simulink model "snap_adc5g_spec_rpi"  (R2019a)
settings: Solver=VariableStepDiscrete  StartTime=0.0  StopTime=10.0  RelTol=1e-3
undefined symbols (not defined in the file): pfb_coeff_gen_calc
libraries: xbsIndex_r4 x13965, casper_library_misc x80, casper_library_delays x43, xps_library x5, xbsReplacements_r4 x2, casper_library_communications x1
(part 3 of 152)

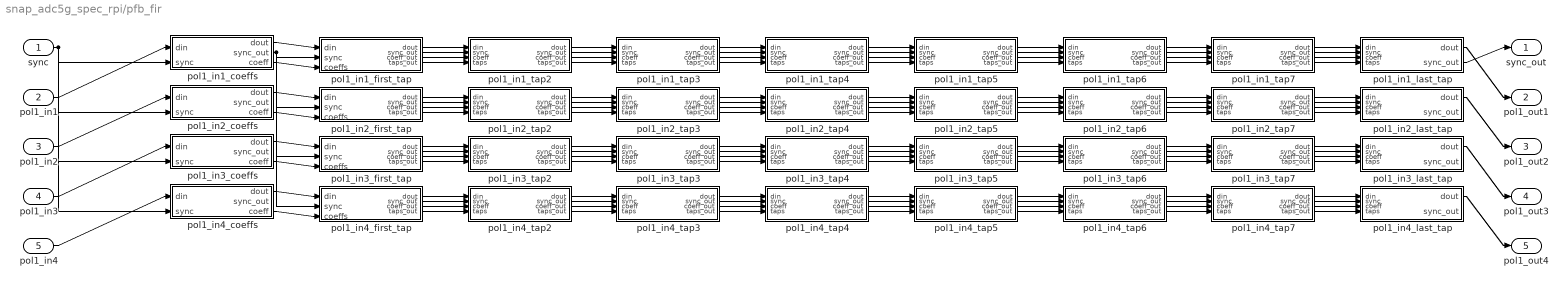
== system snap_adc5g_spec_rpi/pfb_fir ==
  sync : Inport
  pol1_in1 : Inport  Port=2
  pol1_in2 : Inport  Port=3
  pol1_in3 : Inport  Port=4
  pol1_in4 : Inport  Port=5
  pol1_in1_coeffs : Subsystem  AncestorBlock=casper_library_pfbs/pfb_coeff_gen  mask(pfb_coeff_gen){PFBSize=13, CoeffBitWidth=18, TotalTaps=8, CoeffDistMem=off, WindowType=hamming, bram_latency=3, n_inputs=2, nput=0, fwidth=1, debug_mode=off, fan_latency=1}
      mask prompts: PFBSize "Size of PFB: (2^? pnts)"; CoeffBitWidth "Bitwidth of Coefficients:"; TotalTaps "Total Number of Taps:"; CoeffDistMem "Implement Coeff Gen in Distributed Memory"; WindowType "Windowing Function:"; bram_latency "BRAM Latency"; n_inputs "Number of Simultaneous Inputs: (2^?)"; nput "This is input number:"; fwidth "Bin Width (normal=1)"; debug_mode "Debug mode - coeffs are a [1:pfb_size*taps] ramp."; fan_latency "Fanout latency"
      mask init:
      | pfb_coeff_gen_init(gcb, ...
      |     'PFBSize', PFBSize, ...
      |     'CoeffBitWidth', CoeffBitWidth, ...
      |     'TotalTaps', TotalTaps, ...
      |     'CoeffDistMem', CoeffDistMem, ...
      |     'WindowType', WindowType, ...
      |     'bram_latency', bram_latency, ...
      |     'n_inputs', n_inputs, ...
      |     'nput', nput, ...
      |     'fwidth', fwidth, ...
      |     'fan_latency', fan_latency, ...
      |     'debug_mode', debug_mode);
      settings: AttributesFormatString=|
      | PFBSize=13, n_inputs=2,
      | taps=8, input=0
  pol1_in1_first_tap : Subsystem  AncestorBlock=casper_library_pfbs/first_tap  mask(first_tap){PFBSize=13, CoeffBitWidth=18, TotalTaps=8, BitWidthIn=8, WindowType=hamming, mult_latency=2, bram_latency=3, n_inputs=2, fwidth=1, use_hdl=on, use_embedded=off}
      mask prompts: PFBSize "Size of PFB: (2^? pnts)"; CoeffBitWidth "Bitwidth of Coefficients:"; TotalTaps "Total Number of Taps:"; BitWidthIn "Input Bitwidth:"; WindowType "Windowing Function:"; mult_latency "Mult Latency"; bram_latency "BRAM Latency"; n_inputs "Number of Simultaneous Inputs: (2^?)"; fwidth "Bit Width (normal=1)"; use_hdl "Use behavioral HDL for multlipliers"; use_embedded "Use embedded multipliers"
      mask init:
      | first_tap_init(gcb,...
      |     'PFBSize', PFBSize,...
      |     'CoeffBitWidth', CoeffBitWidth,...
      |     'TotalTaps', TotalTaps,...
      |     'BitWidthIn', BitWidthIn,...
      |     'WindowType', WindowType,...
      |     'mult_latency', mult_latency,...
      |     'bram_latency', bram_latency,...
      |     'n_inputs', n_inputs,...
      |     'fwidth', fwidth,...
      |     'use_hdl', use_hdl,...
      |     'use_embedded', use_embedded);
      settings: AttributesFormatString=taps=8
      mask TypeOptions WindowType: bartlett | barthannwin | blackman | blackmanharris | bohamwin | chebwin | flattopwin | gausswin | hamming | hann | kaiser | nuttallwin | parzenwin | rectwin | tukeywin | triang
      mask Callback use_hdl:
      | use_hdl = get_param(gcb,'use_hdl');
      | if( strcmp(use_hdl,'on')),
      |     set_param(gcb, 'use_embedded','off');
      |     set_param(gcb, 'MaskVisibilities',{'on','on','on','on','on','on','on','on','on','on','off'});
      | else,
      |     set_param(gcb, 'MaskVisibilities',{'on','on','on','on','on','on','on','on','on','on','on'});
      | end
  pol1_in1_last_tap : Subsystem  AncestorBlock=casper_library_pfbs/last_tap  mask(last_tap){TotalTaps=8, BitWidthIn=8, BitWidthOut=18, CoeffBitWidth=18, add_latency=1, mult_latency=2, quantization=Round  (unbiased: Even Values), use_hdl=on, use_embedded=off}
      mask prompts: TotalTaps "Total Number of Taps:"; BitWidthIn "Input Bitwidth:"; BitWidthOut "Output Bitwidth:"; CoeffBitWidth "Coeff Bitwidth:"; add_latency "Add Latency"; mult_latency "Mult Latency"; quantization "Quantization Behavior"; use_hdl "Use behavioral HDL for multlipliers"; use_embedded "Use embedded multipliers"
      mask init:
      | last_tap_init(gcb,...
      |     'TotalTaps', TotalTaps,...
      |     'BitWidthIn', BitWidthIn,...
      |     'BitWidthOut', BitWidthOut,...
      |     'CoeffBitWidth', CoeffBitWidth,...
      |     'add_latency', add_latency,...
      |     'mult_latency', mult_latency,...
      |     'quantization', quantization,...
      |     'use_hdl', use_hdl,...
      |     'use_embedded', use_embedded);
      settings: AttributesFormatString=taps=8
      mask TypeOptions quantization: Truncate | Round  (unbiased: +/- Inf) | Round  (unbiased: Even Values)
      mask Callback use_hdl:
      | use_hdl = get_param(gcb,'use_hdl');
      | if( strcmp(use_hdl,'on')),
      |     set_param(gcb, 'use_embedded','off');
      |     set_param(gcb, 'MaskVisibilities',{'on','on','on','on','on','on','on','on','off'});
      | else,
      |     set_param(gcb, 'MaskVisibilities',{'on','on','on','on','on','on','on','on','on'});
      | end
  pol1_in1_tap2 : Subsystem  AncestorBlock=casper_library_pfbs/tap  mask(tap){mult_latency=2, coeff_width=18, coeff_frac_width=17, delay=2048, data_width=8, bram_latency=3, use_hdl=on, use_embedded=off}
      mask prompts: mult_latency "Multiplier Latency"; coeff_width "Coefficient Bit Width In"; coeff_frac_width "Coefficient Fractional Bits"; delay "Data/Sync Delay"; data_width "Data Bit Width In"; bram_latency "BRAM Latency"; use_hdl "Use behavioral HDL for multlipliers"; use_embedded "Use embedded multipliers"
      mask init:
      | use_hdl = get_param(gcb,'use_hdl');
      | use_embedded = get_param(gcb,'use_embedded');
      | set_param(gcb,'LinkStatus','inactive');
      | 
      | set_param([gcb,'/Mult'],'use_embedded',use_embedded);
      | set_param([gcb,'/Mult'],'use_behavioral_HDL',use_hdl);
      | set_param([gcb,'/Mult1'],'use_embedded',use_embedded);
      | set_param([gcb,'/Mult1'],'use_behavioral_HDL',use_hdl);
      mask Callback use_hdl:
      | use_hdl = get_param(gcb,'use_hdl');
      | if( strcmp(use_hdl,'on')),
      |     set_param(gcb, 'use_embedded','off');
      |     set_param(gcb, 'MaskVisibilities',{'on','on','on','on','on','on','on','off'});
      | else,
      |     set_param(gcb, 'MaskVisibilities',{'on','on','on','on','on','on','on','on'});
      | end
  pol1_in1_tap3 : Subsystem  AncestorBlock=casper_library_pfbs/tap  mask(tap){mult_latency=2, coeff_width=18, coeff_frac_width=17, delay=2048, data_width=8, bram_latency=3, use_hdl=on, use_embedded=off}
      mask prompts: mult_latency "Multiplier Latency"; coeff_width "Coefficient Bit Width In"; coeff_frac_width "Coefficient Fractional Bits"; delay "Data/Sync Delay"; data_width "Data Bit Width In"; bram_latency "BRAM Latency"; use_hdl "Use behavioral HDL for multlipliers"; use_embedded "Use embedded multipliers"
      mask init: same as snap_adc5g_spec_rpi/pfb_fir/pol1_in1_tap2
      mask Callback use_hdl:
      | use_hdl = get_param(gcb,'use_hdl');
      | if( strcmp(use_hdl,'on')),
      |     set_param(gcb, 'use_embedded','off');
      |     set_param(gcb, 'MaskVisibilities',{'on','on','on','on','on','on','on','off'});
      | else,
      |     set_param(gcb, 'MaskVisibilities',{'on','on','on','on','on','on','on','on'});
      | end
  pol1_in1_tap4 : Subsystem  AncestorBlock=casper_library_pfbs/tap  mask(tap){mult_latency=2, coeff_width=18, coeff_frac_width=17, delay=2048, data_width=8, bram_latency=3, use_hdl=on, use_embedded=off}
      mask prompts: mult_latency "Multiplier Latency"; coeff_width "Coefficient Bit Width In"; coeff_frac_width "Coefficient Fractional Bits"; delay "Data/Sync Delay"; data_width "Data Bit Width In"; bram_latency "BRAM Latency"; use_hdl "Use behavioral HDL for multlipliers"; use_embedded "Use embedded multipliers"
      mask init: same as snap_adc5g_spec_rpi/pfb_fir/pol1_in1_tap2
      mask Callback use_hdl:
      | use_hdl = get_param(gcb,'use_hdl');
      | if( strcmp(use_hdl,'on')),
      |     set_param(gcb, 'use_embedded','off');
      |     set_param(gcb, 'MaskVisibilities',{'on','on','on','on','on','on','on','off'});
      | else,
      |     set_param(gcb, 'MaskVisibilities',{'on','on','on','on','on','on','on','on'});
      | end
  pol1_in1_tap5 : Subsystem  AncestorBlock=casper_library_pfbs/tap  mask(tap){mult_latency=2, coeff_width=18, coeff_frac_width=17, delay=2048, data_width=8, bram_latency=3, use_hdl=on, use_embedded=off}
      mask prompts: mult_latency "Multiplier Latency"; coeff_width "Coefficient Bit Width In"; coeff_frac_width "Coefficient Fractional Bits"; delay "Data/Sync Delay"; data_width "Data Bit Width In"; bram_latency "BRAM Latency"; use_hdl "Use behavioral HDL for multlipliers"; use_embedded "Use embedded multipliers"
      mask init: same as snap_adc5g_spec_rpi/pfb_fir/pol1_in1_tap2
      mask Callback use_hdl:
      | use_hdl = get_param(gcb,'use_hdl');
      | if( strcmp(use_hdl,'on')),
      |     set_param(gcb, 'use_embedded','off');
      |     set_param(gcb, 'MaskVisibilities',{'on','on','on','on','on','on','on','off'});
      | else,
      |     set_param(gcb, 'MaskVisibilities',{'on','on','on','on','on','on','on','on'});
      | end
  pol1_in1_tap6 : Subsystem  AncestorBlock=casper_library_pfbs/tap  mask(tap){mult_latency=2, coeff_width=18, coeff_frac_width=17, delay=2048, data_width=8, bram_latency=3, use_hdl=on, use_embedded=off}
      mask prompts: mult_latency "Multiplier Latency"; coeff_width "Coefficient Bit Width In"; coeff_frac_width "Coefficient Fractional Bits"; delay "Data/Sync Delay"; data_width "Data Bit Width In"; bram_latency "BRAM Latency"; use_hdl "Use behavioral HDL for multlipliers"; use_embedded "Use embedded multipliers"
      mask init: same as snap_adc5g_spec_rpi/pfb_fir/pol1_in1_tap2
      mask Callback use_hdl:
      | use_hdl = get_param(gcb,'use_hdl');
      | if( strcmp(use_hdl,'on')),
      |     set_param(gcb, 'use_embedded','off');
      |     set_param(gcb, 'MaskVisibilities',{'on','on','on','on','on','on','on','off'});
      | else,
      |     set_param(gcb, 'MaskVisibilities',{'on','on','on','on','on','on','on','on'});
      | end
  pol1_in1_tap7 : Subsystem  AncestorBlock=casper_library_pfbs/tap  mask(tap){mult_latency=2, coeff_width=18, coeff_frac_width=17, delay=2048, data_width=8, bram_latency=3, use_hdl=on, use_embedded=off}
      mask prompts: mult_latency "Multiplier Latency"; coeff_width "Coefficient Bit Width In"; coeff_frac_width "Coefficient Fractional Bits"; delay "Data/Sync Delay"; data_width "Data Bit Width In"; bram_latency "BRAM Latency"; use_hdl "Use behavioral HDL for multlipliers"; use_embedded "Use embedded multipliers"
      mask init: same as snap_adc5g_spec_rpi/pfb_fir/pol1_in1_tap2
      mask Callback use_hdl:
      | use_hdl = get_param(gcb,'use_hdl');
      | if( strcmp(use_hdl,'on')),
      |     set_param(gcb, 'use_embedded','off');
      |     set_param(gcb, 'MaskVisibilities',{'on','on','on','on','on','on','on','off'});
      | else,
      |     set_param(gcb, 'MaskVisibilities',{'on','on','on','on','on','on','on','on'});
      | end
  pol1_in2_coeffs : Subsystem  AncestorBlock=casper_library_pfbs/pfb_coeff_gen  mask(pfb_coeff_gen){PFBSize=13, CoeffBitWidth=18, TotalTaps=8, CoeffDistMem=off, WindowType=hamming, bram_latency=3, n_inputs=2, nput=1, fwidth=1, debug_mode=off, fan_latency=1}
      mask prompts: PFBSize "Size of PFB: (2^? pnts)"; CoeffBitWidth "Bitwidth of Coefficients:"; TotalTaps "Total Number of Taps:"; CoeffDistMem "Implement Coeff Gen in Distributed Memory"; WindowType "Windowing Function:"; bram_latency "BRAM Latency"; n_inputs "Number of Simultaneous Inputs: (2^?)"; nput "This is input number:"; fwidth "Bin Width (normal=1)"; debug_mode "Debug mode - coeffs are a [1:pfb_size*taps] ramp."; fan_latency "Fanout latency"
      mask init: same as snap_adc5g_spec_rpi/pfb_fir/pol1_in1_coeffs
      settings: AttributesFormatString=|
      | PFBSize=13, n_inputs=2,
      | taps=8, input=1
  pol1_in2_first_tap : Subsystem  AncestorBlock=casper_library_pfbs/first_tap  mask(first_tap){PFBSize=13, CoeffBitWidth=18, TotalTaps=8, BitWidthIn=8, WindowType=hamming, mult_latency=2, bram_latency=3, n_inputs=2, fwidth=1, use_hdl=on, use_embedded=off}
      mask prompts: PFBSize "Size of PFB: (2^? pnts)"; CoeffBitWidth "Bitwidth of Coefficients:"; TotalTaps "Total Number of Taps:"; BitWidthIn "Input Bitwidth:"; WindowType "Windowing Function:"; mult_latency "Mult Latency"; bram_latency "BRAM Latency"; n_inputs "Number of Simultaneous Inputs: (2^?)"; fwidth "Bit Width (normal=1)"; use_hdl "Use behavioral HDL for multlipliers"; use_embedded "Use embedded multipliers"
      mask init: same as snap_adc5g_spec_rpi/pfb_fir/pol1_in1_first_tap
      settings: AttributesFormatString=taps=8
      mask TypeOptions WindowType: bartlett | barthannwin | blackman | blackmanharris | bohamwin | chebwin | flattopwin | gausswin | hamming | hann | kaiser | nuttallwin | parzenwin | rectwin | tukeywin | triang
      mask Callback use_hdl:
      | use_hdl = get_param(gcb,'use_hdl');
      | if( strcmp(use_hdl,'on')),
      |     set_param(gcb, 'use_embedded','off');
      |     set_param(gcb, 'MaskVisibilities',{'on','on','on','on','on','on','on','on','on','on','off'});
      | else,
      |     set_param(gcb, 'MaskVisibilities',{'on','on','on','on','on','on','on','on','on','on','on'});
      | end
  pol1_in2_last_tap : Subsystem  AncestorBlock=casper_library_pfbs/last_tap  mask(last_tap){TotalTaps=8, BitWidthIn=8, BitWidthOut=18, CoeffBitWidth=18, add_latency=1, mult_latency=2, quantization=Round  (unbiased: Even Values), use_hdl=on, use_embedded=off}
      mask prompts: TotalTaps "Total Number of Taps:"; BitWidthIn "Input Bitwidth:"; BitWidthOut "Output Bitwidth:"; CoeffBitWidth "Coeff Bitwidth:"; add_latency "Add Latency"; mult_latency "Mult Latency"; quantization "Quantization Behavior"; use_hdl "Use behavioral HDL for multlipliers"; use_embedded "Use embedded multipliers"
      mask init: same as snap_adc5g_spec_rpi/pfb_fir/pol1_in1_last_tap
      settings: AttributesFormatString=taps=8
      mask TypeOptions quantization: Truncate | Round  (unbiased: +/- Inf) | Round  (unbiased: Even Values)
      mask Callback use_hdl:
      | use_hdl = get_param(gcb,'use_hdl');
      | if( strcmp(use_hdl,'on')),
      |     set_param(gcb, 'use_embedded','off');
      |     set_param(gcb, 'MaskVisibilities',{'on','on','on','on','on','on','on','on','off'});
      | else,
      |     set_param(gcb, 'MaskVisibilities',{'on','on','on','on','on','on','on','on','on'});
      | end
  pol1_in2_tap2 : Subsystem  AncestorBlock=casper_library_pfbs/tap  mask(tap){mult_latency=2, coeff_width=18, coeff_frac_width=17, delay=2048, data_width=8, bram_latency=3, use_hdl=on, use_embedded=off}
      mask prompts: mult_latency "Multiplier Latency"; coeff_width "Coefficient Bit Width In"; coeff_frac_width "Coefficient Fractional Bits"; delay "Data/Sync Delay"; data_width "Data Bit Width In"; bram_latency "BRAM Latency"; use_hdl "Use behavioral HDL for multlipliers"; use_embedded "Use embedded multipliers"
      mask init: same as snap_adc5g_spec_rpi/pfb_fir/pol1_in1_tap2
      mask Callback use_hdl:
      | use_hdl = get_param(gcb,'use_hdl');
      | if( strcmp(use_hdl,'on')),
      |     set_param(gcb, 'use_embedded','off');
      |     set_param(gcb, 'MaskVisibilities',{'on','on','on','on','on','on','on','off'});
      | else,
      |     set_param(gcb, 'MaskVisibilities',{'on','on','on','on','on','on','on','on'});
      | end
  pol1_in2_tap3 : Subsystem  AncestorBlock=casper_library_pfbs/tap  mask(tap){mult_latency=2, coeff_width=18, coeff_frac_width=17, delay=2048, data_width=8, bram_latency=3, use_hdl=on, use_embedded=off}
      mask prompts: mult_latency "Multiplier Latency"; coeff_width "Coefficient Bit Width In"; coeff_frac_width "Coefficient Fractional Bits"; delay "Data/Sync Delay"; data_width "Data Bit Width In"; bram_latency "BRAM Latency"; use_hdl "Use behavioral HDL for multlipliers"; use_embedded "Use embedded multipliers"
      mask init: same as snap_adc5g_spec_rpi/pfb_fir/pol1_in1_tap2
      mask Callback use_hdl:
      | use_hdl = get_param(gcb,'use_hdl');
      | if( strcmp(use_hdl,'on')),
      |     set_param(gcb, 'use_embedded','off');
      |     set_param(gcb, 'MaskVisibilities',{'on','on','on','on','on','on','on','off'});
      | else,
      |     set_param(gcb, 'MaskVisibilities',{'on','on','on','on','on','on','on','on'});
      | end
  pol1_in2_tap4 : Subsystem  AncestorBlock=casper_library_pfbs/tap  mask(tap){mult_latency=2, coeff_width=18, coeff_frac_width=17, delay=2048, data_width=8, bram_latency=3, use_hdl=on, use_embedded=off}
      mask prompts: mult_latency "Multiplier Latency"; coeff_width "Coefficient Bit Width In"; coeff_frac_width "Coefficient Fractional Bits"; delay "Data/Sync Delay"; data_width "Data Bit Width In"; bram_latency "BRAM Latency"; use_hdl "Use behavioral HDL for multlipliers"; use_embedded "Use embedded multipliers"
      mask init: same as snap_adc5g_spec_rpi/pfb_fir/pol1_in1_tap2
      mask Callback use_hdl:
      | use_hdl = get_param(gcb,'use_hdl');
      | if( strcmp(use_hdl,'on')),
      |     set_param(gcb, 'use_embedded','off');
      |     set_param(gcb, 'MaskVisibilities',{'on','on','on','on','on','on','on','off'});
      | else,
      |     set_param(gcb, 'MaskVisibilities',{'on','on','on','on','on','on','on','on'});
      | end
  pol1_in2_tap5 : Subsystem  AncestorBlock=casper_library_pfbs/tap  mask(tap){mult_latency=2, coeff_width=18, coeff_frac_width=17, delay=2048, data_width=8, bram_latency=3, use_hdl=on, use_embedded=off}
      mask prompts: mult_latency "Multiplier Latency"; coeff_width "Coefficient Bit Width In"; coeff_frac_width "Coefficient Fractional Bits"; delay "Data/Sync Delay"; data_width "Data Bit Width In"; bram_latency "BRAM Latency"; use_hdl "Use behavioral HDL for multlipliers"; use_embedded "Use embedded multipliers"
      mask init: same as snap_adc5g_spec_rpi/pfb_fir/pol1_in1_tap2
      mask Callback use_hdl:
      | use_hdl = get_param(gcb,'use_hdl');
      | if( strcmp(use_hdl,'on')),
      |     set_param(gcb, 'use_embedded','off');
      |     set_param(gcb, 'MaskVisibilities',{'on','on','on','on','on','on','on','off'});
      | else,
      |     set_param(gcb, 'MaskVisibilities',{'on','on','on','on','on','on','on','on'});
      | end
  pol1_in2_tap6 : Subsystem  AncestorBlock=casper_library_pfbs/tap  mask(tap){mult_latency=2, coeff_width=18, coeff_frac_width=17, delay=2048, data_width=8, bram_latency=3, use_hdl=on, use_embedded=off}
      mask prompts: mult_latency "Multiplier Latency"; coeff_width "Coefficient Bit Width In"; coeff_frac_width "Coefficient Fractional Bits"; delay "Data/Sync Delay"; data_width "Data Bit Width In"; bram_latency "BRAM Latency"; use_hdl "Use behavioral HDL for multlipliers"; use_embedded "Use embedded multipliers"
      mask init: same as snap_adc5g_spec_rpi/pfb_fir/pol1_in1_tap2
      mask Callback use_hdl:
      | use_hdl = get_param(gcb,'use_hdl');
      | if( strcmp(use_hdl,'on')),
      |     set_param(gcb, 'use_embedded','off');
      |     set_param(gcb, 'MaskVisibilities',{'on','on','on','on','on','on','on','off'});
      | else,
      |     set_param(gcb, 'MaskVisibilities',{'on','on','on','on','on','on','on','on'});
      | end
  pol1_in2_tap7 : Subsystem  AncestorBlock=casper_library_pfbs/tap  mask(tap){mult_latency=2, coeff_width=18, coeff_frac_width=17, delay=2048, data_width=8, bram_latency=3, use_hdl=on, use_embedded=off}
      mask prompts: mult_latency "Multiplier Latency"; coeff_width "Coefficient Bit Width In"; coeff_frac_width "Coefficient Fractional Bits"; delay "Data/Sync Delay"; data_width "Data Bit Width In"; bram_latency "BRAM Latency"; use_hdl "Use behavioral HDL for multlipliers"; use_embedded "Use embedded multipliers"
      mask init: same as snap_adc5g_spec_rpi/pfb_fir/pol1_in1_tap2
      mask Callback use_hdl:
      | use_hdl = get_param(gcb,'use_hdl');
      | if( strcmp(use_hdl,'on')),
      |     set_param(gcb, 'use_embedded','off');
      |     set_param(gcb, 'MaskVisibilities',{'on','on','on','on','on','on','on','off'});
      | else,
      |     set_param(gcb, 'MaskVisibilities',{'on','on','on','on','on','on','on','on'});
      | end
  pol1_in3_coeffs : Subsystem  AncestorBlock=casper_library_pfbs/pfb_coeff_gen  mask(pfb_coeff_gen){PFBSize=13, CoeffBitWidth=18, TotalTaps=8, CoeffDistMem=off, WindowType=hamming, bram_latency=3, n_inputs=2, nput=2, fwidth=1, debug_mode=off, fan_latency=1}
      mask prompts: PFBSize "Size of PFB: (2^? pnts)"; CoeffBitWidth "Bitwidth of Coefficients:"; TotalTaps "Total Number of Taps:"; CoeffDistMem "Implement Coeff Gen in Distributed Memory"; WindowType "Windowing Function:"; bram_latency "BRAM Latency"; n_inputs "Number of Simultaneous Inputs: (2^?)"; nput "This is input number:"; fwidth "Bin Width (normal=1)"; debug_mode "Debug mode - coeffs are a [1:pfb_size*taps] ramp."; fan_latency "Fanout latency"
      mask init: same as snap_adc5g_spec_rpi/pfb_fir/pol1_in1_coeffs
      settings: AttributesFormatString=|
      | PFBSize=13, n_inputs=2,
      | taps=8, input=2
  pol1_in3_first_tap : Subsystem  AncestorBlock=casper_library_pfbs/first_tap  mask(first_tap){PFBSize=13, CoeffBitWidth=18, TotalTaps=8, BitWidthIn=8, WindowType=hamming, mult_latency=2, bram_latency=3, n_inputs=2, fwidth=1, use_hdl=on, use_embedded=off}
      mask prompts: PFBSize "Size of PFB: (2^? pnts)"; CoeffBitWidth "Bitwidth of Coefficients:"; TotalTaps "Total Number of Taps:"; BitWidthIn "Input Bitwidth:"; WindowType "Windowing Function:"; mult_latency "Mult Latency"; bram_latency "BRAM Latency"; n_inputs "Number of Simultaneous Inputs: (2^?)"; fwidth "Bit Width (normal=1)"; use_hdl "Use behavioral HDL for multlipliers"; use_embedded "Use embedded multipliers"
      mask init: same as snap_adc5g_spec_rpi/pfb_fir/pol1_in1_first_tap
      settings: AttributesFormatString=taps=8
      mask TypeOptions WindowType: bartlett | barthannwin | blackman | blackmanharris | bohamwin | chebwin | flattopwin | gausswin | hamming | hann | kaiser | nuttallwin | parzenwin | rectwin | tukeywin | triang
      mask Callback use_hdl:
      | use_hdl = get_param(gcb,'use_hdl');
      | if( strcmp(use_hdl,'on')),
      |     set_param(gcb, 'use_embedded','off');
      |     set_param(gcb, 'MaskVisibilities',{'on','on','on','on','on','on','on','on','on','on','off'});
      | else,
      |     set_param(gcb, 'MaskVisibilities',{'on','on','on','on','on','on','on','on','on','on','on'});
      | end
  pol1_in3_last_tap : Subsystem  AncestorBlock=casper_library_pfbs/last_tap  mask(last_tap){TotalTaps=8, BitWidthIn=8, BitWidthOut=18, CoeffBitWidth=18, add_latency=1, mult_latency=2, quantization=Round  (unbiased: Even Values), use_hdl=on, use_embedded=off}
      mask prompts: TotalTaps "Total Number of Taps:"; BitWidthIn "Input Bitwidth:"; BitWidthOut "Output Bitwidth:"; CoeffBitWidth "Coeff Bitwidth:"; add_latency "Add Latency"; mult_latency "Mult Latency"; quantization "Quantization Behavior"; use_hdl "Use behavioral HDL for multlipliers"; use_embedded "Use embedded multipliers"
      mask init: same as snap_adc5g_spec_rpi/pfb_fir/pol1_in1_last_tap
      settings: AttributesFormatString=taps=8
      mask TypeOptions quantization: Truncate | Round  (unbiased: +/- Inf) | Round  (unbiased: Even Values)
      mask Callback use_hdl:
      | use_hdl = get_param(gcb,'use_hdl');
      | if( strcmp(use_hdl,'on')),
      |     set_param(gcb, 'use_embedded','off');
      |     set_param(gcb, 'MaskVisibilities',{'on','on','on','on','on','on','on','on','off'});
      | else,
      |     set_param(gcb, 'MaskVisibilities',{'on','on','on','on','on','on','on','on','on'});
      | end
  pol1_in3_tap2 : Subsystem  AncestorBlock=casper_library_pfbs/tap  mask(tap){mult_latency=2, coeff_width=18, coeff_frac_width=17, delay=2048, data_width=8, bram_latency=3, use_hdl=on, use_embedded=off}
      mask prompts: mult_latency "Multiplier Latency"; coeff_width "Coefficient Bit Width In"; coeff_frac_width "Coefficient Fractional Bits"; delay "Data/Sync Delay"; data_width "Data Bit Width In"; bram_latency "BRAM Latency"; use_hdl "Use behavioral HDL for multlipliers"; use_embedded "Use embedded multipliers"
      mask init: same as snap_adc5g_spec_rpi/pfb_fir/pol1_in1_tap2
      mask Callback use_hdl:
      | use_hdl = get_param(gcb,'use_hdl');
      | if( strcmp(use_hdl,'on')),
      |     set_param(gcb, 'use_embedded','off');
      |     set_param(gcb, 'MaskVisibilities',{'on','on','on','on','on','on','on','off'});
      | else,
      |     set_param(gcb, 'MaskVisibilities',{'on','on','on','on','on','on','on','on'});
      | end
  pol1_in3_tap3 : Subsystem  AncestorBlock=casper_library_pfbs/tap  mask(tap){mult_latency=2, coeff_width=18, coeff_frac_width=17, delay=2048, data_width=8, bram_latency=3, use_hdl=on, use_embedded=off}
      mask prompts: mult_latency "Multiplier Latency"; coeff_width "Coefficient Bit Width In"; coeff_frac_width "Coefficient Fractional Bits"; delay "Data/Sync Delay"; data_width "Data Bit Width In"; bram_latency "BRAM Latency"; use_hdl "Use behavioral HDL for multlipliers"; use_embedded "Use embedded multipliers"
      mask init: same as snap_adc5g_spec_rpi/pfb_fir/pol1_in1_tap2
      mask Callback use_hdl:
      | use_hdl = get_param(gcb,'use_hdl');
      | if( strcmp(use_hdl,'on')),
      |     set_param(gcb, 'use_embedded','off');
      |     set_param(gcb, 'MaskVisibilities',{'on','on','on','on','on','on','on','off'});
      | else,
      |     set_param(gcb, 'MaskVisibilities',{'on','on','on','on','on','on','on','on'});
      | end
  pol1_in3_tap4 : Subsystem  AncestorBlock=casper_library_pfbs/tap  mask(tap){mult_latency=2, coeff_width=18, coeff_frac_width=17, delay=2048, data_width=8, bram_latency=3, use_hdl=on, use_embedded=off}
      mask prompts: mult_latency "Multiplier Latency"; coeff_width "Coefficient Bit Width In"; coeff_frac_width "Coefficient Fractional Bits"; delay "Data/Sync Delay"; data_width "Data Bit Width In"; bram_latency "BRAM Latency"; use_hdl "Use behavioral HDL for multlipliers"; use_embedded "Use embedded multipliers"
      mask init: same as snap_adc5g_spec_rpi/pfb_fir/pol1_in1_tap2
      mask Callback use_hdl:
      | use_hdl = get_param(gcb,'use_hdl');
      | if( strcmp(use_hdl,'on')),
      |     set_param(gcb, 'use_embedded','off');
      |     set_param(gcb, 'MaskVisibilities',{'on','on','on','on','on','on','on','off'});
      | else,
      |     set_param(gcb, 'MaskVisibilities',{'on','on','on','on','on','on','on','on'});
      | end
  pol1_in3_tap5 : Subsystem  AncestorBlock=casper_library_pfbs/tap  mask(tap){mult_latency=2, coeff_width=18, coeff_frac_width=17, delay=2048, data_width=8, bram_latency=3, use_hdl=on, use_embedded=off}
      mask prompts: mult_latency "Multiplier Latency"; coeff_width "Coefficient Bit Width In"; coeff_frac_width "Coefficient Fractional Bits"; delay "Data/Sync Delay"; data_width "Data Bit Width In"; bram_latency "BRAM Latency"; use_hdl "Use behavioral HDL for multlipliers"; use_embedded "Use embedded multipliers"
      mask init: same as snap_adc5g_spec_rpi/pfb_fir/pol1_in1_tap2
      mask Callback use_hdl:
      | use_hdl = get_param(gcb,'use_hdl');
      | if( strcmp(use_hdl,'on')),
      |     set_param(gcb, 'use_embedded','off');
      |     set_param(gcb, 'MaskVisibilities',{'on','on','on','on','on','on','on','off'});
      | else,
      |     set_param(gcb, 'MaskVisibilities',{'on','on','on','on','on','on','on','on'});
      | end
  pol1_in3_tap6 : Subsystem  AncestorBlock=casper_library_pfbs/tap  mask(tap){mult_latency=2, coeff_width=18, coeff_frac_width=17, delay=2048, data_width=8, bram_latency=3, use_hdl=on, use_embedded=off}
      mask prompts: mult_latency "Multiplier Latency"; coeff_width "Coefficient Bit Width In"; coeff_frac_width "Coefficient Fractional Bits"; delay "Data/Sync Delay"; data_width "Data Bit Width In"; bram_latency "BRAM Latency"; use_hdl "Use behavioral HDL for multlipliers"; use_embedded "Use embedded multipliers"
      mask init: same as snap_adc5g_spec_rpi/pfb_fir/pol1_in1_tap2
      mask Callback use_hdl:
      | use_hdl = get_param(gcb,'use_hdl');
      | if( strcmp(use_hdl,'on')),
      |     set_param(gcb, 'use_embedded','off');
      |     set_param(gcb, 'MaskVisibilities',{'on','on','on','on','on','on','on','off'});
      | else,
      |     set_param(gcb, 'MaskVisibilities',{'on','on','on','on','on','on','on','on'});
      | end
  pol1_in3_tap7 : Subsystem  AncestorBlock=casper_library_pfbs/tap  mask(tap){mult_latency=2, coeff_width=18, coeff_frac_width=17, delay=2048, data_width=8, bram_latency=3, use_hdl=on, use_embedded=off}
      mask prompts: mult_latency "Multiplier Latency"; coeff_width "Coefficient Bit Width In"; coeff_frac_width "Coefficient Fractional Bits"; delay "Data/Sync Delay"; data_width "Data Bit Width In"; bram_latency "BRAM Latency"; use_hdl "Use behavioral HDL for multlipliers"; use_embedded "Use embedded multipliers"
      mask init: same as snap_adc5g_spec_rpi/pfb_fir/pol1_in1_tap2
      mask Callback use_hdl:
      | use_hdl = get_param(gcb,'use_hdl');
      | if( strcmp(use_hdl,'on')),
      |     set_param(gcb, 'use_embedded','off');
      |     set_param(gcb, 'MaskVisibilities',{'on','on','on','on','on','on','on','off'});
      | else,
      |     set_param(gcb, 'MaskVisibilities',{'on','on','on','on','on','on','on','on'});
      | end
  pol1_in4_coeffs : Subsystem  AncestorBlock=casper_library_pfbs/pfb_coeff_gen  mask(pfb_coeff_gen){PFBSize=13, CoeffBitWidth=18, TotalTaps=8, CoeffDistMem=off, WindowType=hamming, bram_latency=3, n_inputs=2, nput=3, fwidth=1, debug_mode=off, fan_latency=1}
      mask prompts: PFBSize "Size of PFB: (2^? pnts)"; CoeffBitWidth "Bitwidth of Coefficients:"; TotalTaps "Total Number of Taps:"; CoeffDistMem "Implement Coeff Gen in Distributed Memory"; WindowType "Windowing Function:"; bram_latency "BRAM Latency"; n_inputs "Number of Simultaneous Inputs: (2^?)"; nput "This is input number:"; fwidth "Bin Width (normal=1)"; debug_mode "Debug mode - coeffs are a [1:pfb_size*taps] ramp."; fan_latency "Fanout latency"
      mask init: same as snap_adc5g_spec_rpi/pfb_fir/pol1_in1_coeffs
      settings: AttributesFormatString=|
      | PFBSize=13, n_inputs=2,
      | taps=8, input=3
  pol1_in4_first_tap : Subsystem  AncestorBlock=casper_library_pfbs/first_tap  mask(first_tap){PFBSize=13, CoeffBitWidth=18, TotalTaps=8, BitWidthIn=8, WindowType=hamming, mult_latency=2, bram_latency=3, n_inputs=2, fwidth=1, use_hdl=on, use_embedded=off}
      mask prompts: PFBSize "Size of PFB: (2^? pnts)"; CoeffBitWidth "Bitwidth of Coefficients:"; TotalTaps "Total Number of Taps:"; BitWidthIn "Input Bitwidth:"; WindowType "Windowing Function:"; mult_latency "Mult Latency"; bram_latency "BRAM Latency"; n_inputs "Number of Simultaneous Inputs: (2^?)"; fwidth "Bit Width (normal=1)"; use_hdl "Use behavioral HDL for multlipliers"; use_embedded "Use embedded multipliers"
      mask init: same as snap_adc5g_spec_rpi/pfb_fir/pol1_in1_first_tap
      settings: AttributesFormatString=taps=8
      mask TypeOptions WindowType: bartlett | barthannwin | blackman | blackmanharris | bohamwin | chebwin | flattopwin | gausswin | hamming | hann | kaiser | nuttallwin | parzenwin | rectwin | tukeywin | triang
      mask Callback use_hdl:
      | use_hdl = get_param(gcb,'use_hdl');
      | if( strcmp(use_hdl,'on')),
      |     set_param(gcb, 'use_embedded','off');
      |     set_param(gcb, 'MaskVisibilities',{'on','on','on','on','on','on','on','on','on','on','off'});
      | else,
      |     set_param(gcb, 'MaskVisibilities',{'on','on','on','on','on','on','on','on','on','on','on'});
      | end
  pol1_in4_last_tap : Subsystem  AncestorBlock=casper_library_pfbs/last_tap  mask(last_tap){TotalTaps=8, BitWidthIn=8, BitWidthOut=18, CoeffBitWidth=18, add_latency=1, mult_latency=2, quantization=Round  (unbiased: Even Values), use_hdl=on, use_embedded=off}
      mask prompts: TotalTaps "Total Number of Taps:"; BitWidthIn "Input Bitwidth:"; BitWidthOut "Output Bitwidth:"; CoeffBitWidth "Coeff Bitwidth:"; add_latency "Add Latency"; mult_latency "Mult Latency"; quantization "Quantization Behavior"; use_hdl "Use behavioral HDL for multlipliers"; use_embedded "Use embedded multipliers"
      mask init: same as snap_adc5g_spec_rpi/pfb_fir/pol1_in1_last_tap
      settings: AttributesFormatString=taps=8
      mask TypeOptions quantization: Truncate | Round  (unbiased: +/- Inf) | Round  (unbiased: Even Values)
      mask Callback use_hdl:
      | use_hdl = get_param(gcb,'use_hdl');
      | if( strcmp(use_hdl,'on')),
      |     set_param(gcb, 'use_embedded','off');
      |     set_param(gcb, 'MaskVisibilities',{'on','on','on','on','on','on','on','on','off'});
      | else,
      |     set_param(gcb, 'MaskVisibilities',{'on','on','on','on','on','on','on','on','on'});
      | end
  pol1_in4_tap2 : Subsystem  AncestorBlock=casper_library_pfbs/tap  mask(tap){mult_latency=2, coeff_width=18, coeff_frac_width=17, delay=2048, data_width=8, bram_latency=3, use_hdl=on, use_embedded=off}
      mask prompts: mult_latency "Multiplier Latency"; coeff_width "Coefficient Bit Width In"; coeff_frac_width "Coefficient Fractional Bits"; delay "Data/Sync Delay"; data_width "Data Bit Width In"; bram_latency "BRAM Latency"; use_hdl "Use behavioral HDL for multlipliers"; use_embedded "Use embedded multipliers"
      mask init: same as snap_adc5g_spec_rpi/pfb_fir/pol1_in1_tap2
      mask Callback use_hdl:
      | use_hdl = get_param(gcb,'use_hdl');
      | if( strcmp(use_hdl,'on')),
      |     set_param(gcb, 'use_embedded','off');
      |     set_param(gcb, 'MaskVisibilities',{'on','on','on','on','on','on','on','off'});
      | else,
      |     set_param(gcb, 'MaskVisibilities',{'on','on','on','on','on','on','on','on'});
      | end
  pol1_in4_tap3 : Subsystem  AncestorBlock=casper_library_pfbs/tap  mask(tap){mult_latency=2, coeff_width=18, coeff_frac_width=17, delay=2048, data_width=8, bram_latency=3, use_hdl=on, use_embedded=off}
      mask prompts: mult_latency "Multiplier Latency"; coeff_width "Coefficient Bit Width In"; coeff_frac_width "Coefficient Fractional Bits"; delay "Data/Sync Delay"; data_width "Data Bit Width In"; bram_latency "BRAM Latency"; use_hdl "Use behavioral HDL for multlipliers"; use_embedded "Use embedded multipliers"
      mask init: same as snap_adc5g_spec_rpi/pfb_fir/pol1_in1_tap2
      mask Callback use_hdl:
      | use_hdl = get_param(gcb,'use_hdl');
      | if( strcmp(use_hdl,'on')),
      |     set_param(gcb, 'use_embedded','off');
      |     set_param(gcb, 'MaskVisibilities',{'on','on','on','on','on','on','on','off'});
      | else,
      |     set_param(gcb, 'MaskVisibilities',{'on','on','on','on','on','on','on','on'});
      | end
  pol1_in4_tap4 : Subsystem  AncestorBlock=casper_library_pfbs/tap  mask(tap){mult_latency=2, coeff_width=18, coeff_frac_width=17, delay=2048, data_width=8, bram_latency=3, use_hdl=on, use_embedded=off}
      mask prompts: mult_latency "Multiplier Latency"; coeff_width "Coefficient Bit Width In"; coeff_frac_width "Coefficient Fractional Bits"; delay "Data/Sync Delay"; data_width "Data Bit Width In"; bram_latency "BRAM Latency"; use_hdl "Use behavioral HDL for multlipliers"; use_embedded "Use embedded multipliers"
      mask init: same as snap_adc5g_spec_rpi/pfb_fir/pol1_in1_tap2
      mask Callback use_hdl:
      | use_hdl = get_param(gcb,'use_hdl');
      | if( strcmp(use_hdl,'on')),
      |     set_param(gcb, 'use_embedded','off');
      |     set_param(gcb, 'MaskVisibilities',{'on','on','on','on','on','on','on','off'});
      | else,
      |     set_param(gcb, 'MaskVisibilities',{'on','on','on','on','on','on','on','on'});
      | end
  pol1_in4_tap5 : Subsystem  AncestorBlock=casper_library_pfbs/tap  mask(tap){mult_latency=2, coeff_width=18, coeff_frac_width=17, delay=2048, data_width=8, bram_latency=3, use_hdl=on, use_embedded=off}
      mask prompts: mult_latency "Multiplier Latency"; coeff_width "Coefficient Bit Width In"; coeff_frac_width "Coefficient Fractional Bits"; delay "Data/Sync Delay"; data_width "Data Bit Width In"; bram_latency "BRAM Latency"; use_hdl "Use behavioral HDL for multlipliers"; use_embedded "Use embedded multipliers"
      mask init: same as snap_adc5g_spec_rpi/pfb_fir/pol1_in1_tap2
      mask Callback use_hdl:
      | use_hdl = get_param(gcb,'use_hdl');
      | if( strcmp(use_hdl,'on')),
      |     set_param(gcb, 'use_embedded','off');
      |     set_param(gcb, 'MaskVisibilities',{'on','on','on','on','on','on','on','off'});
      | else,
      |     set_param(gcb, 'MaskVisibilities',{'on','on','on','on','on','on','on','on'});
      | end
  pol1_in4_tap6 : Subsystem  AncestorBlock=casper_library_pfbs/tap  mask(tap){mult_latency=2, coeff_width=18, coeff_frac_width=17, delay=2048, data_width=8, bram_latency=3, use_hdl=on, use_embedded=off}
      mask prompts: mult_latency "Multiplier Latency"; coeff_width "Coefficient Bit Width In"; coeff_frac_width "Coefficient Fractional Bits"; delay "Data/Sync Delay"; data_width "Data Bit Width In"; bram_latency "BRAM Latency"; use_hdl "Use behavioral HDL for multlipliers"; use_embedded "Use embedded multipliers"
      mask init: same as snap_adc5g_spec_rpi/pfb_fir/pol1_in1_tap2
      mask Callback use_hdl:
      | use_hdl = get_param(gcb,'use_hdl');
      | if( strcmp(use_hdl,'on')),
      |     set_param(gcb, 'use_embedded','off');
      |     set_param(gcb, 'MaskVisibilities',{'on','on','on','on','on','on','on','off'});
      | else,
      |     set_param(gcb, 'MaskVisibilities',{'on','on','on','on','on','on','on','on'});
      | end
  pol1_in4_tap7 : Subsystem  AncestorBlock=casper_library_pfbs/tap  mask(tap){mult_latency=2, coeff_width=18, coeff_frac_width=17, delay=2048, data_width=8, bram_latency=3, use_hdl=on, use_embedded=off}
      mask prompts: mult_latency "Multiplier Latency"; coeff_width "Coefficient Bit Width In"; coeff_frac_width "Coefficient Fractional Bits"; delay "Data/Sync Delay"; data_width "Data Bit Width In"; bram_latency "BRAM Latency"; use_hdl "Use behavioral HDL for multlipliers"; use_embedded "Use embedded multipliers"
      mask init: same as snap_adc5g_spec_rpi/pfb_fir/pol1_in1_tap2
      mask Callback use_hdl:
      | use_hdl = get_param(gcb,'use_hdl');
      | if( strcmp(use_hdl,'on')),
      |     set_param(gcb, 'use_embedded','off');
      |     set_param(gcb, 'MaskVisibilities',{'on','on','on','on','on','on','on','off'});
      | else,
      |     set_param(gcb, 'MaskVisibilities',{'on','on','on','on','on','on','on','on'});
      | end
  sync_out : Outport
  pol1_out1 : Outport  Port=2
  pol1_out2 : Outport  Port=3
  pol1_out3 : Outport  Port=4
  pol1_out4 : Outport  Port=5
  wires:
  pol1_in1/1 -> pol1_in1_coeffs/1(din)
  sync/1 -> pol1_in1_coeffs/2(sync), pol1_in2_coeffs/2(sync), pol1_in3_coeffs/2(sync), pol1_in4_coeffs/2(sync)
  pol1_in1_coeffs/1(dout) -> pol1_in1_first_tap/1(din)
  pol1_in1_coeffs/2(sync_out) -> pol1_in1_first_tap/2(sync), pol1_in2_first_tap/2(sync), pol1_in3_first_tap/2(sync), pol1_in4_first_tap/2(sync)
  pol1_in1_coeffs/3(coeff) -> pol1_in1_first_tap/3(coeffs)
  pol1_in1_first_tap/1(dout) -> pol1_in1_tap2/1(din)
  pol1_in1_first_tap/2(sync_out) -> pol1_in1_tap2/2(sync)
  pol1_in1_first_tap/3(coeff_out) -> pol1_in1_tap2/3(coeff)
  pol1_in1_first_tap/4(taps_out) -> pol1_in1_tap2/4(taps)
  pol1_in1_tap2/1(dout) -> pol1_in1_tap3/1(din)
  pol1_in1_tap2/2(sync_out) -> pol1_in1_tap3/2(sync)
  pol1_in1_tap2/3(coeff_out) -> pol1_in1_tap3/3(coeff)
  pol1_in1_tap2/4(taps_out) -> pol1_in1_tap3/4(taps)
  pol1_in1_tap3/1(dout) -> pol1_in1_tap4/1(din)
  pol1_in1_tap3/2(sync_out) -> pol1_in1_tap4/2(sync)
  pol1_in1_tap3/3(coeff_out) -> pol1_in1_tap4/3(coeff)
  pol1_in1_tap3/4(taps_out) -> pol1_in1_tap4/4(taps)
  pol1_in1_tap4/1(dout) -> pol1_in1_tap5/1(din)
  pol1_in1_tap4/2(sync_out) -> pol1_in1_tap5/2(sync)
  pol1_in1_tap4/3(coeff_out) -> pol1_in1_tap5/3(coeff)
  pol1_in1_tap4/4(taps_out) -> pol1_in1_tap5/4(taps)
  pol1_in1_tap5/1(dout) -> pol1_in1_tap6/1(din)
  pol1_in1_tap5/2(sync_out) -> pol1_in1_tap6/2(sync)
  pol1_in1_tap5/3(coeff_out) -> pol1_in1_tap6/3(coeff)
  pol1_in1_tap5/4(taps_out) -> pol1_in1_tap6/4(taps)
  pol1_in1_tap6/1(dout) -> pol1_in1_tap7/1(din)
  pol1_in1_tap6/2(sync_out) -> pol1_in1_tap7/2(sync)
  pol1_in1_tap6/3(coeff_out) -> pol1_in1_tap7/3(coeff)
  pol1_in1_tap6/4(taps_out) -> pol1_in1_tap7/4(taps)
  pol1_in1_tap7/1(dout) -> pol1_in1_last_tap/1(din)
  pol1_in1_tap7/2(sync_out) -> pol1_in1_last_tap/2(sync)
  pol1_in1_tap7/3(coeff_out) -> pol1_in1_last_tap/3(coeff)
  pol1_in1_tap7/4(taps_out) -> pol1_in1_last_tap/4(taps)
  pol1_in1_last_tap/1(dout) -> pol1_out1/1
  pol1_in1_last_tap/2(sync_out) -> sync_out/1
  pol1_in2/1 -> pol1_in2_coeffs/1(din)
  pol1_in2_coeffs/1(dout) -> pol1_in2_first_tap/1(din)
  pol1_in2_coeffs/3(coeff) -> pol1_in2_first_tap/3(coeffs)
  pol1_in2_first_tap/1(dout) -> pol1_in2_tap2/1(din)
  pol1_in2_first_tap/2(sync_out) -> pol1_in2_tap2/2(sync)
  pol1_in2_first_tap/3(coeff_out) -> pol1_in2_tap2/3(coeff)
  pol1_in2_first_tap/4(taps_out) -> pol1_in2_tap2/4(taps)
  pol1_in2_tap2/1(dout) -> pol1_in2_tap3/1(din)
  pol1_in2_tap2/2(sync_out) -> pol1_in2_tap3/2(sync)
  pol1_in2_tap2/3(coeff_out) -> pol1_in2_tap3/3(coeff)
  pol1_in2_tap2/4(taps_out) -> pol1_in2_tap3/4(taps)
  pol1_in2_tap3/1(dout) -> pol1_in2_tap4/1(din)
  pol1_in2_tap3/2(sync_out) -> pol1_in2_tap4/2(sync)
  pol1_in2_tap3/3(coeff_out) -> pol1_in2_tap4/3(coeff)
  pol1_in2_tap3/4(taps_out) -> pol1_in2_tap4/4(taps)
  pol1_in2_tap4/1(dout) -> pol1_in2_tap5/1(din)
  pol1_in2_tap4/2(sync_out) -> pol1_in2_tap5/2(sync)
  pol1_in2_tap4/3(coeff_out) -> pol1_in2_tap5/3(coeff)
  pol1_in2_tap4/4(taps_out) -> pol1_in2_tap5/4(taps)
  pol1_in2_tap5/1(dout) -> pol1_in2_tap6/1(din)
  pol1_in2_tap5/2(sync_out) -> pol1_in2_tap6/2(sync)
  pol1_in2_tap5/3(coeff_out) -> pol1_in2_tap6/3(coeff)
  pol1_in2_tap5/4(taps_out) -> pol1_in2_tap6/4(taps)
  pol1_in2_tap6/1(dout) -> pol1_in2_tap7/1(din)
  pol1_in2_tap6/2(sync_out) -> pol1_in2_tap7/2(sync)
  pol1_in2_tap6/3(coeff_out) -> pol1_in2_tap7/3(coeff)
  pol1_in2_tap6/4(taps_out) -> pol1_in2_tap7/4(taps)
  pol1_in2_tap7/1(dout) -> pol1_in2_last_tap/1(din)
  pol1_in2_tap7/2(sync_out) -> pol1_in2_last_tap/2(sync)
  pol1_in2_tap7/3(coeff_out) -> pol1_in2_last_tap/3(coeff)
  pol1_in2_tap7/4(taps_out) -> pol1_in2_last_tap/4(taps)
  pol1_in2_last_tap/1(dout) -> pol1_out2/1
  pol1_in3/1 -> pol1_in3_coeffs/1(din)
  pol1_in3_coeffs/1(dout) -> pol1_in3_first_tap/1(din)
  pol1_in3_coeffs/3(coeff) -> pol1_in3_first_tap/3(coeffs)
  pol1_in3_first_tap/1(dout) -> pol1_in3_tap2/1(din)
  pol1_in3_first_tap/2(sync_out) -> pol1_in3_tap2/2(sync)
  pol1_in3_first_tap/3(coeff_out) -> pol1_in3_tap2/3(coeff)
  pol1_in3_first_tap/4(taps_out) -> pol1_in3_tap2/4(taps)
  pol1_in3_tap2/1(dout) -> pol1_in3_tap3/1(din)
  pol1_in3_tap2/2(sync_out) -> pol1_in3_tap3/2(sync)
  pol1_in3_tap2/3(coeff_out) -> pol1_in3_tap3/3(coeff)
  pol1_in3_tap2/4(taps_out) -> pol1_in3_tap3/4(taps)
  pol1_in3_tap3/1(dout) -> pol1_in3_tap4/1(din)
  pol1_in3_tap3/2(sync_out) -> pol1_in3_tap4/2(sync)
  pol1_in3_tap3/3(coeff_out) -> pol1_in3_tap4/3(coeff)
  pol1_in3_tap3/4(taps_out) -> pol1_in3_tap4/4(taps)
  pol1_in3_tap4/1(dout) -> pol1_in3_tap5/1(din)
  pol1_in3_tap4/2(sync_out) -> pol1_in3_tap5/2(sync)
  pol1_in3_tap4/3(coeff_out) -> pol1_in3_tap5/3(coeff)
  pol1_in3_tap4/4(taps_out) -> pol1_in3_tap5/4(taps)
  pol1_in3_tap5/1(dout) -> pol1_in3_tap6/1(din)
  pol1_in3_tap5/2(sync_out) -> pol1_in3_tap6/2(sync)
  pol1_in3_tap5/3(coeff_out) -> pol1_in3_tap6/3(coeff)
  pol1_in3_tap5/4(taps_out) -> pol1_in3_tap6/4(taps)
  pol1_in3_tap6/1(dout) -> pol1_in3_tap7/1(din)
  pol1_in3_tap6/2(sync_out) -> pol1_in3_tap7/2(sync)
  pol1_in3_tap6/3(coeff_out) -> pol1_in3_tap7/3(coeff)
  pol1_in3_tap6/4(taps_out) -> pol1_in3_tap7/4(taps)
  pol1_in3_tap7/1(dout) -> pol1_in3_last_tap/1(din)
  pol1_in3_tap7/2(sync_out) -> pol1_in3_last_tap/2(sync)
  pol1_in3_tap7/3(coeff_out) -> pol1_in3_last_tap/3(coeff)
  pol1_in3_tap7/4(taps_out) -> pol1_in3_last_tap/4(taps)
  pol1_in3_last_tap/1(dout) -> pol1_out3/1
  pol1_in4/1 -> pol1_in4_coeffs/1(din)
  pol1_in4_coeffs/1(dout) -> pol1_in4_first_tap/1(din)
  pol1_in4_coeffs/3(coeff) -> pol1_in4_first_tap/3(coeffs)
  pol1_in4_first_tap/1(dout) -> pol1_in4_tap2/1(din)
  pol1_in4_first_tap/2(sync_out) -> pol1_in4_tap2/2(sync)
  pol1_in4_first_tap/3(coeff_out) -> pol1_in4_tap2/3(coeff)
  pol1_in4_first_tap/4(taps_out) -> pol1_in4_tap2/4(taps)
  pol1_in4_tap2/1(dout) -> pol1_in4_tap3/1(din)
  pol1_in4_tap2/2(sync_out) -> pol1_in4_tap3/2(sync)
  pol1_in4_tap2/3(coeff_out) -> pol1_in4_tap3/3(coeff)
  pol1_in4_tap2/4(taps_out) -> pol1_in4_tap3/4(taps)
  pol1_in4_tap3/1(dout) -> pol1_in4_tap4/1(din)
  pol1_in4_tap3/2(sync_out) -> pol1_in4_tap4/2(sync)
  pol1_in4_tap3/3(coeff_out) -> pol1_in4_tap4/3(coeff)
  pol1_in4_tap3/4(taps_out) -> pol1_in4_tap4/4(taps)
  pol1_in4_tap4/1(dout) -> pol1_in4_tap5/1(din)
  pol1_in4_tap4/2(sync_out) -> pol1_in4_tap5/2(sync)
  pol1_in4_tap4/3(coeff_out) -> pol1_in4_tap5/3(coeff)
  pol1_in4_tap4/4(taps_out) -> pol1_in4_tap5/4(taps)
  pol1_in4_tap5/1(dout) -> pol1_in4_tap6/1(din)
  pol1_in4_tap5/2(sync_out) -> pol1_in4_tap6/2(sync)
  pol1_in4_tap5/3(coeff_out) -> pol1_in4_tap6/3(coeff)
  pol1_in4_tap5/4(taps_out) -> pol1_in4_tap6/4(taps)
  pol1_in4_tap6/1(dout) -> pol1_in4_tap7/1(din)
  pol1_in4_tap6/2(sync_out) -> pol1_in4_tap7/2(sync)
  pol1_in4_tap6/3(coeff_out) -> pol1_in4_tap7/3(coeff)
  pol1_in4_tap6/4(taps_out) -> pol1_in4_tap7/4(taps)
  pol1_in4_tap7/1(dout) -> pol1_in4_last_tap/1(din)
  pol1_in4_tap7/2(sync_out) -> pol1_in4_last_tap/2(sync)
  pol1_in4_tap7/3(coeff_out) -> pol1_in4_last_tap/3(coeff)
  pol1_in4_tap7/4(taps_out) -> pol1_in4_last_tap/4(taps)
  pol1_in4_last_tap/1(dout) -> pol1_out4/1
